simulink model "dc_motor_open_loop"  (R2025b)
settings: Solver=ode45  StartTime=0.0  StopTime=8  MaxStep=0.002  RelTol=1e-7  AbsTol=1e-9
model workspace (MAT data in the model file):
  J = 0.01
  Ke = 0.1
  Kt = 0.1
  L = 0.01
  R = 1
  Udc = 12
  b = 0.001
  loadTorque = 0
settings Model: Creator=alosw  LastModifiedBy=alosw

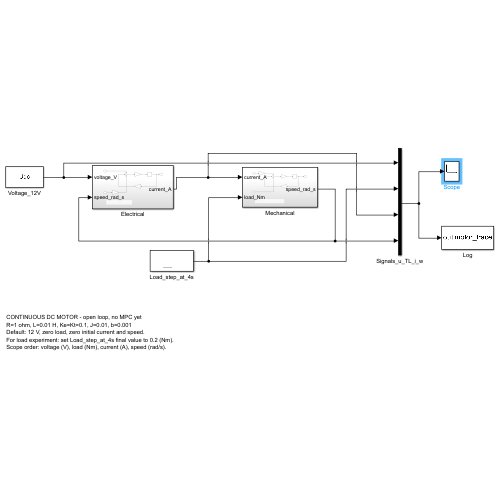
[thumbnail: Simulink's stored preview of the top-level diagram]
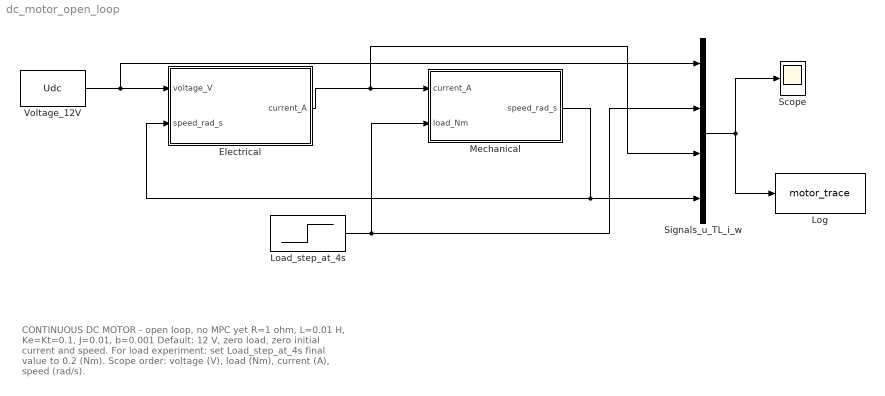
== system dc_motor_open_loop ==
  note: CONTINUOUS DC MOTOR - open loop, no MPC yet
      | R=1 ohm, L=0.01 H, Ke=Kt=0.1, J=0.01, b=0.001
      | Default: 12 V, zero load, zero initial current and speed.
      | For load experiment: set Load_step_at_4s final value to 0.2 (Nm).
      | Scope order: voltage (V), load (Nm), current (A), speed (rad/s).
  Electrical : Subsystem
  Load_step_at_4s : Step  Time=4  After=loadTorque  SampleTime=0
  Log : ToWorkspace  VariableName=motor_trace  SaveFormat=Timeseries  SampleTime=-1
  Mechanical : Subsystem
  Scope : Scope
      settings: ActiveDisplayYMinimum=2.0049179158663648  ActiveDisplayYMaximum=98.902354108012275
  Signals_u_TL_i_w : Mux
  Voltage_12V : Constant  Value=Udc
  wires:
  Voltage_12V/1 -> Signals_u_TL_i_w/1, Electrical/1(voltage_V)
  Electrical/1(current_A) -> Signals_u_TL_i_w/3, Mechanical/1(current_A)
  Mechanical/1(speed_rad_s) -> Electrical/2(speed_rad_s), Signals_u_TL_i_w/4
  Load_step_at_4s/1 -> Signals_u_TL_i_w/2, Mechanical/2(load_Nm)
  Signals_u_TL_i_w/1 -> Log/1, Scope/1

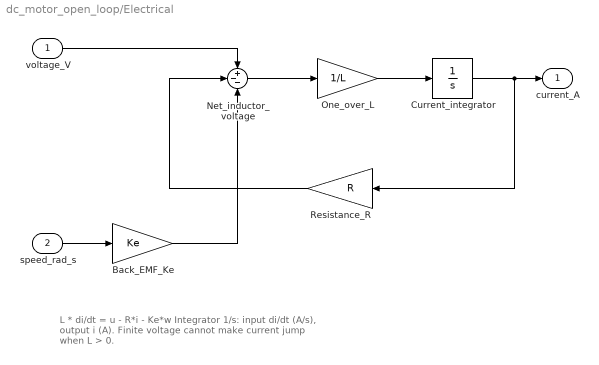
== system dc_motor_open_loop/Electrical ==
  note: L * di/dt = u - R*i - Ke*w
      | Integrator 1/s: input di/dt (A/s), output i (A).
      | Finite voltage cannot make current jump when L > 0.
  voltage_V : Inport
  speed_rad_s : Inport  Port=2
  Back_EMF_Ke : Gain  Gain=Ke
  Current_integrator : Integrator
  Net_inductor_voltage : Sum  Inputs=+--
  One_over_L : Gain  Gain=1/L
  Resistance_R : Gain  Gain=R
  current_A : Outport
  wires:
  voltage_V/1 -> Net_inductor_voltage/1
  Resistance_R/1 -> Net_inductor_voltage/2
  Back_EMF_Ke/1 -> Net_inductor_voltage/3
  Net_inductor_voltage/1 -> One_over_L/1
  One_over_L/1 -> Current_integrator/1
  Current_integrator/1 -> current_A/1, Resistance_R/1
  speed_rad_s/1 -> Back_EMF_Ke/1

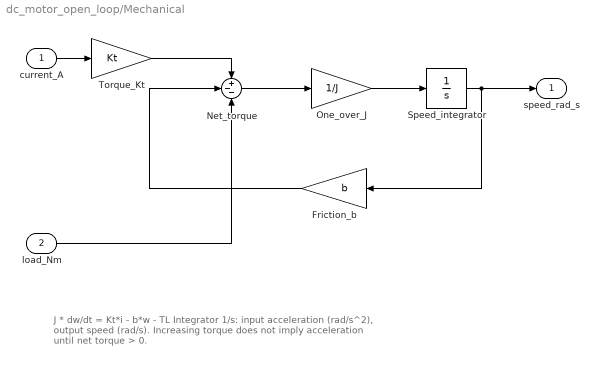
== system dc_motor_open_loop/Mechanical ==
  note: J * dw/dt = Kt*i - b*w - TL
      | Integrator 1/s: input acceleration (rad/s^2), output speed (rad/s).
      | Increasing torque does not imply acceleration until net torque > 0.
  current_A : Inport
  load_Nm : Inport  Port=2
  Friction_b : Gain  Gain=b
  Net_torque : Sum  Inputs=+--
  One_over_J : Gain  Gain=1/J
  Speed_integrator : Integrator
  Torque_Kt : Gain  Gain=Kt
  speed_rad_s : Outport
  wires:
  current_A/1 -> Torque_Kt/1
  Torque_Kt/1 -> Net_torque/1
  Friction_b/1 -> Net_torque/2
  load_Nm/1 -> Net_torque/3
  Net_torque/1 -> One_over_J/1
  One_over_J/1 -> Speed_integrator/1
  Speed_integrator/1 -> speed_rad_s/1, Friction_b/1
